simulink model "TB32_A25R_ClampMix"  (R2025a)
settings: Solver=FixedStepDiscrete  StartTime=0  StopTime=TB.t_end  FixedStep=TB.dt  RelTol=1e-3
InitFcn:
  | % 모델과 같은 폴더의 초기화 스크립트를 실행해 P(설계 파라미터)와 TB(시험 조건)를 만든다.
  | run(fullfile(fileparts(get_param(bdroot, 'FileName')), 'TB32_init.m'));
values from neighbouring files (symbols this model uses):
  TB = struct()    [TB32_init.m]    (also in run_TB32.m = evalin('base', 'TB'))
libraries: fl_lib x227, nesl_utility x83
(part 4 of 4)

== system TB32_A25R_ClampMix/StageA_Module3/StageA_Phase6/S2_A_VOUT ==
  note: 스위치 셀: 이상 스위치(R_on, G_off) + 역병렬 바디 다이오드(Vf, R_d) + 출력용량 C_oss
      | 게이트: 전역 태그 "gA_P6_S2" (> 0.5 이면 도통)
  C_oss : fl_lib/Electrical/Electrical Elements/Capacitor  c=Coss F  r=1e-6 Ohm  g=0 1/Ohm  i_specify=off  i_priority=None  i=0 A  i_nominal_specify=off  i_nominal_value=1  i_nominal_unit=A  v_specify=off  v_priority=None  v=0 V  v_nominal_specify=off  v_nominal_value=1  v_nominal_unit=V  vc_specify=off  vc_priority=High  vc=0 V  vc_nominal_specify=off  vc_nominal_value=1  vc_nominal_unit=V
  D_body : fl_lib/Electrical/Electrical Elements/Diode  Vf=Vf V  Ron=Rd Ohm  Goff=Goffd 1/Ohm  i_specify=off  i_priority=None  i=0 A  i_nominal_specify=off  i_nominal_value=1  i_nominal_unit=A  v_specify=off  v_priority=None  v=0 V  v_nominal_specify=off  v_nominal_value=1  v_nominal_unit=V
  Gate_PS : nesl_utility/Simulink-PS Converter  PhysicalDomain=network_engine_domain  SubClassName=ps_input  LeftPortType=input  RightPortType=output  PseudoPeriodic=off  Frequencies=[]  NoiseDistribution=none  NoiseParameters=[]  Unit=1  AffineConversion=off  FilteringAndDerivatives=zero  SimscapeFilterOrder=1  InputFilterTimeConstant=0.001  UdotUserProvided=0
  SW : fl_lib/Electrical/Electrical Elements/Switch  R_closed=Ron Ohm  G_open=Goff 1/Ohm  Threshold=0.5  i_specify=off  i_priority=None  i=0 A  i_nominal_specify=off  i_nominal_value=1  i_nominal_unit=A  v_specify=off  v_priority=None  v=0 V  v_nominal_specify=off  v_nominal_value=1  v_nominal_unit=V
  D : PMIOPort  Side=Left
  S : PMIOPort  Port=2  Side=Right
  wires:
  [gA_P6_S2] -> Gate_PS/1
  connections:
  Gate_PS/RConn1 -- SW/RConn1
  SW/LConn1 -- D/RConn1 -- D_body/RConn1 -- C_oss/LConn1
  SW/RConn2 -- D_body/LConn1 -- S/RConn1 -- C_oss/RConn1

== system TB32_A25R_ClampMix/StageA_Module3/StageA_Phase6/S3_VOUT_B ==
  note: 스위치 셀: 이상 스위치(R_on, G_off) + 역병렬 바디 다이오드(Vf, R_d) + 출력용량 C_oss
      | 게이트: 전역 태그 "gA_P6_S3" (> 0.5 이면 도통)
  C_oss : fl_lib/Electrical/Electrical Elements/Capacitor  c=Coss F  r=1e-6 Ohm  g=0 1/Ohm  i_specify=off  i_priority=None  i=0 A  i_nominal_specify=off  i_nominal_value=1  i_nominal_unit=A  v_specify=off  v_priority=None  v=0 V  v_nominal_specify=off  v_nominal_value=1  v_nominal_unit=V  vc_specify=off  vc_priority=High  vc=0 V  vc_nominal_specify=off  vc_nominal_value=1  vc_nominal_unit=V
  D_body : fl_lib/Electrical/Electrical Elements/Diode  Vf=Vf V  Ron=Rd Ohm  Goff=Goffd 1/Ohm  i_specify=off  i_priority=None  i=0 A  i_nominal_specify=off  i_nominal_value=1  i_nominal_unit=A  v_specify=off  v_priority=None  v=0 V  v_nominal_specify=off  v_nominal_value=1  v_nominal_unit=V
  Gate_PS : nesl_utility/Simulink-PS Converter  PhysicalDomain=network_engine_domain  SubClassName=ps_input  LeftPortType=input  RightPortType=output  PseudoPeriodic=off  Frequencies=[]  NoiseDistribution=none  NoiseParameters=[]  Unit=1  AffineConversion=off  FilteringAndDerivatives=zero  SimscapeFilterOrder=1  InputFilterTimeConstant=0.001  UdotUserProvided=0
  SW : fl_lib/Electrical/Electrical Elements/Switch  R_closed=Ron Ohm  G_open=Goff 1/Ohm  Threshold=0.5  i_specify=off  i_priority=None  i=0 A  i_nominal_specify=off  i_nominal_value=1  i_nominal_unit=A  v_specify=off  v_priority=None  v=0 V  v_nominal_specify=off  v_nominal_value=1  v_nominal_unit=V
  D : PMIOPort  Side=Left
  S : PMIOPort  Port=2  Side=Right
  wires:
  [gA_P6_S3] -> Gate_PS/1
  connections:
  Gate_PS/RConn1 -- SW/RConn1
  SW/LConn1 -- D/RConn1 -- D_body/RConn1 -- C_oss/LConn1
  SW/RConn2 -- D_body/LConn1 -- S/RConn1 -- C_oss/RConn1

== system TB32_A25R_ClampMix/StageA_Module3/StageA_Phase6/S4_B_GND ==
  note: 스위치 셀: 이상 스위치(R_on, G_off) + 역병렬 바디 다이오드(Vf, R_d) + 출력용량 C_oss
      | 게이트: 전역 태그 "gA_P6_S4" (> 0.5 이면 도통)
  C_oss : fl_lib/Electrical/Electrical Elements/Capacitor  c=Coss F  r=1e-6 Ohm  g=0 1/Ohm  i_specify=off  i_priority=None  i=0 A  i_nominal_specify=off  i_nominal_value=1  i_nominal_unit=A  v_specify=off  v_priority=None  v=0 V  v_nominal_specify=off  v_nominal_value=1  v_nominal_unit=V  vc_specify=off  vc_priority=High  vc=0 V  vc_nominal_specify=off  vc_nominal_value=1  vc_nominal_unit=V
  D_body : fl_lib/Electrical/Electrical Elements/Diode  Vf=Vf V  Ron=Rd Ohm  Goff=Goffd 1/Ohm  i_specify=off  i_priority=None  i=0 A  i_nominal_specify=off  i_nominal_value=1  i_nominal_unit=A  v_specify=off  v_priority=None  v=0 V  v_nominal_specify=off  v_nominal_value=1  v_nominal_unit=V
  Gate_PS : nesl_utility/Simulink-PS Converter  PhysicalDomain=network_engine_domain  SubClassName=ps_input  LeftPortType=input  RightPortType=output  PseudoPeriodic=off  Frequencies=[]  NoiseDistribution=none  NoiseParameters=[]  Unit=1  AffineConversion=off  FilteringAndDerivatives=zero  SimscapeFilterOrder=1  InputFilterTimeConstant=0.001  UdotUserProvided=0
  SW : fl_lib/Electrical/Electrical Elements/Switch  R_closed=Ron Ohm  G_open=Goff 1/Ohm  Threshold=0.5  i_specify=off  i_priority=None  i=0 A  i_nominal_specify=off  i_nominal_value=1  i_nominal_unit=A  v_specify=off  v_priority=None  v=0 V  v_nominal_specify=off  v_nominal_value=1  v_nominal_unit=V
  D : PMIOPort  Side=Left
  S : PMIOPort  Port=2  Side=Right
  wires:
  [gA_P6_S4] -> Gate_PS/1
  connections:
  Gate_PS/RConn1 -- SW/RConn1
  SW/LConn1 -- D/RConn1 -- D_body/RConn1 -- C_oss/LConn1
  SW/RConn2 -- D_body/LConn1 -- S/RConn1 -- C_oss/RConn1

== system TB32_A25R_ClampMix/StageA_Module4/StageA_Phase7/S1_VIN_A ==
  note: 스위치 셀: 이상 스위치(R_on, G_off) + 역병렬 바디 다이오드(Vf, R_d) + 출력용량 C_oss
      | 게이트: 전역 태그 "gA_P7_S1" (> 0.5 이면 도통)
  C_oss : fl_lib/Electrical/Electrical Elements/Capacitor  c=Coss F  r=1e-6 Ohm  g=0 1/Ohm  i_specify=off  i_priority=None  i=0 A  i_nominal_specify=off  i_nominal_value=1  i_nominal_unit=A  v_specify=off  v_priority=None  v=0 V  v_nominal_specify=off  v_nominal_value=1  v_nominal_unit=V  vc_specify=off  vc_priority=High  vc=0 V  vc_nominal_specify=off  vc_nominal_value=1  vc_nominal_unit=V
  D_body : fl_lib/Electrical/Electrical Elements/Diode  Vf=Vf V  Ron=Rd Ohm  Goff=Goffd 1/Ohm  i_specify=off  i_priority=None  i=0 A  i_nominal_specify=off  i_nominal_value=1  i_nominal_unit=A  v_specify=off  v_priority=None  v=0 V  v_nominal_specify=off  v_nominal_value=1  v_nominal_unit=V
  Gate_PS : nesl_utility/Simulink-PS Converter  PhysicalDomain=network_engine_domain  SubClassName=ps_input  LeftPortType=input  RightPortType=output  PseudoPeriodic=off  Frequencies=[]  NoiseDistribution=none  NoiseParameters=[]  Unit=1  AffineConversion=off  FilteringAndDerivatives=zero  SimscapeFilterOrder=1  InputFilterTimeConstant=0.001  UdotUserProvided=0
  SW : fl_lib/Electrical/Electrical Elements/Switch  R_closed=Ron Ohm  G_open=Goff 1/Ohm  Threshold=0.5  i_specify=off  i_priority=None  i=0 A  i_nominal_specify=off  i_nominal_value=1  i_nominal_unit=A  v_specify=off  v_priority=None  v=0 V  v_nominal_specify=off  v_nominal_value=1  v_nominal_unit=V
  D : PMIOPort  Side=Left
  S : PMIOPort  Port=2  Side=Right
  wires:
  [gA_P7_S1] -> Gate_PS/1
  connections:
  Gate_PS/RConn1 -- SW/RConn1
  SW/LConn1 -- D/RConn1 -- D_body/RConn1 -- C_oss/LConn1
  SW/RConn2 -- D_body/LConn1 -- S/RConn1 -- C_oss/RConn1

== system TB32_A25R_ClampMix/StageA_Module4/StageA_Phase7/S2_A_VOUT ==
  note: 스위치 셀: 이상 스위치(R_on, G_off) + 역병렬 바디 다이오드(Vf, R_d) + 출력용량 C_oss
      | 게이트: 전역 태그 "gA_P7_S2" (> 0.5 이면 도통)
  C_oss : fl_lib/Electrical/Electrical Elements/Capacitor  c=Coss F  r=1e-6 Ohm  g=0 1/Ohm  i_specify=off  i_priority=None  i=0 A  i_nominal_specify=off  i_nominal_value=1  i_nominal_unit=A  v_specify=off  v_priority=None  v=0 V  v_nominal_specify=off  v_nominal_value=1  v_nominal_unit=V  vc_specify=off  vc_priority=High  vc=0 V  vc_nominal_specify=off  vc_nominal_value=1  vc_nominal_unit=V
  D_body : fl_lib/Electrical/Electrical Elements/Diode  Vf=Vf V  Ron=Rd Ohm  Goff=Goffd 1/Ohm  i_specify=off  i_priority=None  i=0 A  i_nominal_specify=off  i_nominal_value=1  i_nominal_unit=A  v_specify=off  v_priority=None  v=0 V  v_nominal_specify=off  v_nominal_value=1  v_nominal_unit=V
  Gate_PS : nesl_utility/Simulink-PS Converter  PhysicalDomain=network_engine_domain  SubClassName=ps_input  LeftPortType=input  RightPortType=output  PseudoPeriodic=off  Frequencies=[]  NoiseDistribution=none  NoiseParameters=[]  Unit=1  AffineConversion=off  FilteringAndDerivatives=zero  SimscapeFilterOrder=1  InputFilterTimeConstant=0.001  UdotUserProvided=0
  SW : fl_lib/Electrical/Electrical Elements/Switch  R_closed=Ron Ohm  G_open=Goff 1/Ohm  Threshold=0.5  i_specify=off  i_priority=None  i=0 A  i_nominal_specify=off  i_nominal_value=1  i_nominal_unit=A  v_specify=off  v_priority=None  v=0 V  v_nominal_specify=off  v_nominal_value=1  v_nominal_unit=V
  D : PMIOPort  Side=Left
  S : PMIOPort  Port=2  Side=Right
  wires:
  [gA_P7_S2] -> Gate_PS/1
  connections:
  Gate_PS/RConn1 -- SW/RConn1
  SW/LConn1 -- D/RConn1 -- D_body/RConn1 -- C_oss/LConn1
  SW/RConn2 -- D_body/LConn1 -- S/RConn1 -- C_oss/RConn1

== system TB32_A25R_ClampMix/StageA_Module4/StageA_Phase7/S3_VOUT_B ==
  note: 스위치 셀: 이상 스위치(R_on, G_off) + 역병렬 바디 다이오드(Vf, R_d) + 출력용량 C_oss
      | 게이트: 전역 태그 "gA_P7_S3" (> 0.5 이면 도통)
  C_oss : fl_lib/Electrical/Electrical Elements/Capacitor  c=Coss F  r=1e-6 Ohm  g=0 1/Ohm  i_specify=off  i_priority=None  i=0 A  i_nominal_specify=off  i_nominal_value=1  i_nominal_unit=A  v_specify=off  v_priority=None  v=0 V  v_nominal_specify=off  v_nominal_value=1  v_nominal_unit=V  vc_specify=off  vc_priority=High  vc=0 V  vc_nominal_specify=off  vc_nominal_value=1  vc_nominal_unit=V
  D_body : fl_lib/Electrical/Electrical Elements/Diode  Vf=Vf V  Ron=Rd Ohm  Goff=Goffd 1/Ohm  i_specify=off  i_priority=None  i=0 A  i_nominal_specify=off  i_nominal_value=1  i_nominal_unit=A  v_specify=off  v_priority=None  v=0 V  v_nominal_specify=off  v_nominal_value=1  v_nominal_unit=V
  Gate_PS : nesl_utility/Simulink-PS Converter  PhysicalDomain=network_engine_domain  SubClassName=ps_input  LeftPortType=input  RightPortType=output  PseudoPeriodic=off  Frequencies=[]  NoiseDistribution=none  NoiseParameters=[]  Unit=1  AffineConversion=off  FilteringAndDerivatives=zero  SimscapeFilterOrder=1  InputFilterTimeConstant=0.001  UdotUserProvided=0
  SW : fl_lib/Electrical/Electrical Elements/Switch  R_closed=Ron Ohm  G_open=Goff 1/Ohm  Threshold=0.5  i_specify=off  i_priority=None  i=0 A  i_nominal_specify=off  i_nominal_value=1  i_nominal_unit=A  v_specify=off  v_priority=None  v=0 V  v_nominal_specify=off  v_nominal_value=1  v_nominal_unit=V
  D : PMIOPort  Side=Left
  S : PMIOPort  Port=2  Side=Right
  wires:
  [gA_P7_S3] -> Gate_PS/1
  connections:
  Gate_PS/RConn1 -- SW/RConn1
  SW/LConn1 -- D/RConn1 -- D_body/RConn1 -- C_oss/LConn1
  SW/RConn2 -- D_body/LConn1 -- S/RConn1 -- C_oss/RConn1

== system TB32_A25R_ClampMix/StageA_Module4/StageA_Phase7/S4_B_GND ==
  note: 스위치 셀: 이상 스위치(R_on, G_off) + 역병렬 바디 다이오드(Vf, R_d) + 출력용량 C_oss
      | 게이트: 전역 태그 "gA_P7_S4" (> 0.5 이면 도통)
  C_oss : fl_lib/Electrical/Electrical Elements/Capacitor  c=Coss F  r=1e-6 Ohm  g=0 1/Ohm  i_specify=off  i_priority=None  i=0 A  i_nominal_specify=off  i_nominal_value=1  i_nominal_unit=A  v_specify=off  v_priority=None  v=0 V  v_nominal_specify=off  v_nominal_value=1  v_nominal_unit=V  vc_specify=off  vc_priority=High  vc=0 V  vc_nominal_specify=off  vc_nominal_value=1  vc_nominal_unit=V
  D_body : fl_lib/Electrical/Electrical Elements/Diode  Vf=Vf V  Ron=Rd Ohm  Goff=Goffd 1/Ohm  i_specify=off  i_priority=None  i=0 A  i_nominal_specify=off  i_nominal_value=1  i_nominal_unit=A  v_specify=off  v_priority=None  v=0 V  v_nominal_specify=off  v_nominal_value=1  v_nominal_unit=V
  Gate_PS : nesl_utility/Simulink-PS Converter  PhysicalDomain=network_engine_domain  SubClassName=ps_input  LeftPortType=input  RightPortType=output  PseudoPeriodic=off  Frequencies=[]  NoiseDistribution=none  NoiseParameters=[]  Unit=1  AffineConversion=off  FilteringAndDerivatives=zero  SimscapeFilterOrder=1  InputFilterTimeConstant=0.001  UdotUserProvided=0
  SW : fl_lib/Electrical/Electrical Elements/Switch  R_closed=Ron Ohm  G_open=Goff 1/Ohm  Threshold=0.5  i_specify=off  i_priority=None  i=0 A  i_nominal_specify=off  i_nominal_value=1  i_nominal_unit=A  v_specify=off  v_priority=None  v=0 V  v_nominal_specify=off  v_nominal_value=1  v_nominal_unit=V
  D : PMIOPort  Side=Left
  S : PMIOPort  Port=2  Side=Right
  wires:
  [gA_P7_S4] -> Gate_PS/1
  connections:
  Gate_PS/RConn1 -- SW/RConn1
  SW/LConn1 -- D/RConn1 -- D_body/RConn1 -- C_oss/LConn1
  SW/RConn2 -- D_body/LConn1 -- S/RConn1 -- C_oss/RConn1

== system TB32_A25R_ClampMix/StageA_Module4/StageA_Phase8/S1_VIN_A ==
  note: 스위치 셀: 이상 스위치(R_on, G_off) + 역병렬 바디 다이오드(Vf, R_d) + 출력용량 C_oss
      | 게이트: 전역 태그 "gA_P8_S1" (> 0.5 이면 도통)
  C_oss : fl_lib/Electrical/Electrical Elements/Capacitor  c=Coss F  r=1e-6 Ohm  g=0 1/Ohm  i_specify=off  i_priority=None  i=0 A  i_nominal_specify=off  i_nominal_value=1  i_nominal_unit=A  v_specify=off  v_priority=None  v=0 V  v_nominal_specify=off  v_nominal_value=1  v_nominal_unit=V  vc_specify=off  vc_priority=High  vc=0 V  vc_nominal_specify=off  vc_nominal_value=1  vc_nominal_unit=V
  D_body : fl_lib/Electrical/Electrical Elements/Diode  Vf=Vf V  Ron=Rd Ohm  Goff=Goffd 1/Ohm  i_specify=off  i_priority=None  i=0 A  i_nominal_specify=off  i_nominal_value=1  i_nominal_unit=A  v_specify=off  v_priority=None  v=0 V  v_nominal_specify=off  v_nominal_value=1  v_nominal_unit=V
  Gate_PS : nesl_utility/Simulink-PS Converter  PhysicalDomain=network_engine_domain  SubClassName=ps_input  LeftPortType=input  RightPortType=output  PseudoPeriodic=off  Frequencies=[]  NoiseDistribution=none  NoiseParameters=[]  Unit=1  AffineConversion=off  FilteringAndDerivatives=zero  SimscapeFilterOrder=1  InputFilterTimeConstant=0.001  UdotUserProvided=0
  SW : fl_lib/Electrical/Electrical Elements/Switch  R_closed=Ron Ohm  G_open=Goff 1/Ohm  Threshold=0.5  i_specify=off  i_priority=None  i=0 A  i_nominal_specify=off  i_nominal_value=1  i_nominal_unit=A  v_specify=off  v_priority=None  v=0 V  v_nominal_specify=off  v_nominal_value=1  v_nominal_unit=V
  D : PMIOPort  Side=Left
  S : PMIOPort  Port=2  Side=Right
  wires:
  [gA_P8_S1] -> Gate_PS/1
  connections:
  Gate_PS/RConn1 -- SW/RConn1
  SW/LConn1 -- D/RConn1 -- D_body/RConn1 -- C_oss/LConn1
  SW/RConn2 -- D_body/LConn1 -- S/RConn1 -- C_oss/RConn1

== system TB32_A25R_ClampMix/StageA_Module4/StageA_Phase8/S2_A_VOUT ==
  note: 스위치 셀: 이상 스위치(R_on, G_off) + 역병렬 바디 다이오드(Vf, R_d) + 출력용량 C_oss
      | 게이트: 전역 태그 "gA_P8_S2" (> 0.5 이면 도통)
  C_oss : fl_lib/Electrical/Electrical Elements/Capacitor  c=Coss F  r=1e-6 Ohm  g=0 1/Ohm  i_specify=off  i_priority=None  i=0 A  i_nominal_specify=off  i_nominal_value=1  i_nominal_unit=A  v_specify=off  v_priority=None  v=0 V  v_nominal_specify=off  v_nominal_value=1  v_nominal_unit=V  vc_specify=off  vc_priority=High  vc=0 V  vc_nominal_specify=off  vc_nominal_value=1  vc_nominal_unit=V
  D_body : fl_lib/Electrical/Electrical Elements/Diode  Vf=Vf V  Ron=Rd Ohm  Goff=Goffd 1/Ohm  i_specify=off  i_priority=None  i=0 A  i_nominal_specify=off  i_nominal_value=1  i_nominal_unit=A  v_specify=off  v_priority=None  v=0 V  v_nominal_specify=off  v_nominal_value=1  v_nominal_unit=V
  Gate_PS : nesl_utility/Simulink-PS Converter  PhysicalDomain=network_engine_domain  SubClassName=ps_input  LeftPortType=input  RightPortType=output  PseudoPeriodic=off  Frequencies=[]  NoiseDistribution=none  NoiseParameters=[]  Unit=1  AffineConversion=off  FilteringAndDerivatives=zero  SimscapeFilterOrder=1  InputFilterTimeConstant=0.001  UdotUserProvided=0
  SW : fl_lib/Electrical/Electrical Elements/Switch  R_closed=Ron Ohm  G_open=Goff 1/Ohm  Threshold=0.5  i_specify=off  i_priority=None  i=0 A  i_nominal_specify=off  i_nominal_value=1  i_nominal_unit=A  v_specify=off  v_priority=None  v=0 V  v_nominal_specify=off  v_nominal_value=1  v_nominal_unit=V
  D : PMIOPort  Side=Left
  S : PMIOPort  Port=2  Side=Right
  wires:
  [gA_P8_S2] -> Gate_PS/1
  connections:
  Gate_PS/RConn1 -- SW/RConn1
  SW/LConn1 -- D/RConn1 -- D_body/RConn1 -- C_oss/LConn1
  SW/RConn2 -- D_body/LConn1 -- S/RConn1 -- C_oss/RConn1

== system TB32_A25R_ClampMix/StageA_Module4/StageA_Phase8/S3_VOUT_B ==
  note: 스위치 셀: 이상 스위치(R_on, G_off) + 역병렬 바디 다이오드(Vf, R_d) + 출력용량 C_oss
      | 게이트: 전역 태그 "gA_P8_S3" (> 0.5 이면 도통)
  C_oss : fl_lib/Electrical/Electrical Elements/Capacitor  c=Coss F  r=1e-6 Ohm  g=0 1/Ohm  i_specify=off  i_priority=None  i=0 A  i_nominal_specify=off  i_nominal_value=1  i_nominal_unit=A  v_specify=off  v_priority=None  v=0 V  v_nominal_specify=off  v_nominal_value=1  v_nominal_unit=V  vc_specify=off  vc_priority=High  vc=0 V  vc_nominal_specify=off  vc_nominal_value=1  vc_nominal_unit=V
  D_body : fl_lib/Electrical/Electrical Elements/Diode  Vf=Vf V  Ron=Rd Ohm  Goff=Goffd 1/Ohm  i_specify=off  i_priority=None  i=0 A  i_nominal_specify=off  i_nominal_value=1  i_nominal_unit=A  v_specify=off  v_priority=None  v=0 V  v_nominal_specify=off  v_nominal_value=1  v_nominal_unit=V
  Gate_PS : nesl_utility/Simulink-PS Converter  PhysicalDomain=network_engine_domain  SubClassName=ps_input  LeftPortType=input  RightPortType=output  PseudoPeriodic=off  Frequencies=[]  NoiseDistribution=none  NoiseParameters=[]  Unit=1  AffineConversion=off  FilteringAndDerivatives=zero  SimscapeFilterOrder=1  InputFilterTimeConstant=0.001  UdotUserProvided=0
  SW : fl_lib/Electrical/Electrical Elements/Switch  R_closed=Ron Ohm  G_open=Goff 1/Ohm  Threshold=0.5  i_specify=off  i_priority=None  i=0 A  i_nominal_specify=off  i_nominal_value=1  i_nominal_unit=A  v_specify=off  v_priority=None  v=0 V  v_nominal_specify=off  v_nominal_value=1  v_nominal_unit=V
  D : PMIOPort  Side=Left
  S : PMIOPort  Port=2  Side=Right
  wires:
  [gA_P8_S3] -> Gate_PS/1
  connections:
  Gate_PS/RConn1 -- SW/RConn1
  SW/LConn1 -- D/RConn1 -- D_body/RConn1 -- C_oss/LConn1
  SW/RConn2 -- D_body/LConn1 -- S/RConn1 -- C_oss/RConn1

== system TB32_A25R_ClampMix/StageA_Module4/StageA_Phase8/S4_B_GND ==
  note: 스위치 셀: 이상 스위치(R_on, G_off) + 역병렬 바디 다이오드(Vf, R_d) + 출력용량 C_oss
      | 게이트: 전역 태그 "gA_P8_S4" (> 0.5 이면 도통)
  C_oss : fl_lib/Electrical/Electrical Elements/Capacitor  c=Coss F  r=1e-6 Ohm  g=0 1/Ohm  i_specify=off  i_priority=None  i=0 A  i_nominal_specify=off  i_nominal_value=1  i_nominal_unit=A  v_specify=off  v_priority=None  v=0 V  v_nominal_specify=off  v_nominal_value=1  v_nominal_unit=V  vc_specify=off  vc_priority=High  vc=0 V  vc_nominal_specify=off  vc_nominal_value=1  vc_nominal_unit=V
  D_body : fl_lib/Electrical/Electrical Elements/Diode  Vf=Vf V  Ron=Rd Ohm  Goff=Goffd 1/Ohm  i_specify=off  i_priority=None  i=0 A  i_nominal_specify=off  i_nominal_value=1  i_nominal_unit=A  v_specify=off  v_priority=None  v=0 V  v_nominal_specify=off  v_nominal_value=1  v_nominal_unit=V
  Gate_PS : nesl_utility/Simulink-PS Converter  PhysicalDomain=network_engine_domain  SubClassName=ps_input  LeftPortType=input  RightPortType=output  PseudoPeriodic=off  Frequencies=[]  NoiseDistribution=none  NoiseParameters=[]  Unit=1  AffineConversion=off  FilteringAndDerivatives=zero  SimscapeFilterOrder=1  InputFilterTimeConstant=0.001  UdotUserProvided=0
  SW : fl_lib/Electrical/Electrical Elements/Switch  R_closed=Ron Ohm  G_open=Goff 1/Ohm  Threshold=0.5  i_specify=off  i_priority=None  i=0 A  i_nominal_specify=off  i_nominal_value=1  i_nominal_unit=A  v_specify=off  v_priority=None  v=0 V  v_nominal_specify=off  v_nominal_value=1  v_nominal_unit=V
  D : PMIOPort  Side=Left
  S : PMIOPort  Port=2  Side=Right
  wires:
  [gA_P8_S4] -> Gate_PS/1
  connections:
  Gate_PS/RConn1 -- SW/RConn1
  SW/LConn1 -- D/RConn1 -- D_body/RConn1 -- C_oss/LConn1
  SW/RConn2 -- D_body/LConn1 -- S/RConn1 -- C_oss/RConn1

== system TB32_A25R_ClampMix/StageC_Regulated/Primary_Bridge/Q1_leg1_high ==
  note: 스위치 셀: 이상 스위치(R_on, G_off) + 역병렬 바디 다이오드(Vf, R_d) + 출력용량 C_oss
      | 게이트: 전역 태그 "gC_Q1" (> 0.5 이면 도통)
  C_oss : fl_lib/Electrical/Electrical Elements/Capacitor  c=Coss F  r=1e-6 Ohm  g=0 1/Ohm  i_specify=off  i_priority=None  i=0 A  i_nominal_specify=off  i_nominal_value=1  i_nominal_unit=A  v_specify=off  v_priority=None  v=0 V  v_nominal_specify=off  v_nominal_value=1  v_nominal_unit=V  vc_specify=off  vc_priority=High  vc=0 V  vc_nominal_specify=off  vc_nominal_value=1  vc_nominal_unit=V
  D_body : fl_lib/Electrical/Electrical Elements/Diode  Vf=Vf V  Ron=Rd Ohm  Goff=Goffd 1/Ohm  i_specify=off  i_priority=None  i=0 A  i_nominal_specify=off  i_nominal_value=1  i_nominal_unit=A  v_specify=off  v_priority=None  v=0 V  v_nominal_specify=off  v_nominal_value=1  v_nominal_unit=V
  Gate_PS : nesl_utility/Simulink-PS Converter  PhysicalDomain=network_engine_domain  SubClassName=ps_input  LeftPortType=input  RightPortType=output  PseudoPeriodic=off  Frequencies=[]  NoiseDistribution=none  NoiseParameters=[]  Unit=1  AffineConversion=off  FilteringAndDerivatives=zero  SimscapeFilterOrder=1  InputFilterTimeConstant=0.001  UdotUserProvided=0
  SW : fl_lib/Electrical/Electrical Elements/Switch  R_closed=Ron Ohm  G_open=Goff 1/Ohm  Threshold=0.5  i_specify=off  i_priority=None  i=0 A  i_nominal_specify=off  i_nominal_value=1  i_nominal_unit=A  v_specify=off  v_priority=None  v=0 V  v_nominal_specify=off  v_nominal_value=1  v_nominal_unit=V
  D : PMIOPort  Side=Left
  S : PMIOPort  Port=2  Side=Right
  wires:
  [gC_Q1] -> Gate_PS/1
  connections:
  Gate_PS/RConn1 -- SW/RConn1
  SW/LConn1 -- D/RConn1 -- D_body/RConn1 -- C_oss/LConn1
  SW/RConn2 -- D_body/LConn1 -- S/RConn1 -- C_oss/RConn1

== system TB32_A25R_ClampMix/StageC_Regulated/Primary_Bridge/Q2_leg1_low ==
  note: 스위치 셀: 이상 스위치(R_on, G_off) + 역병렬 바디 다이오드(Vf, R_d) + 출력용량 C_oss
      | 게이트: 전역 태그 "gC_Q2" (> 0.5 이면 도통)
  C_oss : fl_lib/Electrical/Electrical Elements/Capacitor  c=Coss F  r=1e-6 Ohm  g=0 1/Ohm  i_specify=off  i_priority=None  i=0 A  i_nominal_specify=off  i_nominal_value=1  i_nominal_unit=A  v_specify=off  v_priority=None  v=0 V  v_nominal_specify=off  v_nominal_value=1  v_nominal_unit=V  vc_specify=off  vc_priority=High  vc=0 V  vc_nominal_specify=off  vc_nominal_value=1  vc_nominal_unit=V
  D_body : fl_lib/Electrical/Electrical Elements/Diode  Vf=Vf V  Ron=Rd Ohm  Goff=Goffd 1/Ohm  i_specify=off  i_priority=None  i=0 A  i_nominal_specify=off  i_nominal_value=1  i_nominal_unit=A  v_specify=off  v_priority=None  v=0 V  v_nominal_specify=off  v_nominal_value=1  v_nominal_unit=V
  Gate_PS : nesl_utility/Simulink-PS Converter  PhysicalDomain=network_engine_domain  SubClassName=ps_input  LeftPortType=input  RightPortType=output  PseudoPeriodic=off  Frequencies=[]  NoiseDistribution=none  NoiseParameters=[]  Unit=1  AffineConversion=off  FilteringAndDerivatives=zero  SimscapeFilterOrder=1  InputFilterTimeConstant=0.001  UdotUserProvided=0
  SW : fl_lib/Electrical/Electrical Elements/Switch  R_closed=Ron Ohm  G_open=Goff 1/Ohm  Threshold=0.5  i_specify=off  i_priority=None  i=0 A  i_nominal_specify=off  i_nominal_value=1  i_nominal_unit=A  v_specify=off  v_priority=None  v=0 V  v_nominal_specify=off  v_nominal_value=1  v_nominal_unit=V
  D : PMIOPort  Side=Left
  S : PMIOPort  Port=2  Side=Right
  wires:
  [gC_Q2] -> Gate_PS/1
  connections:
  Gate_PS/RConn1 -- SW/RConn1
  SW/LConn1 -- D/RConn1 -- D_body/RConn1 -- C_oss/LConn1
  SW/RConn2 -- D_body/LConn1 -- S/RConn1 -- C_oss/RConn1

== system TB32_A25R_ClampMix/StageC_Regulated/Primary_Bridge/Q3_leg2_high ==
  note: 스위치 셀: 이상 스위치(R_on, G_off) + 역병렬 바디 다이오드(Vf, R_d) + 출력용량 C_oss
      | 게이트: 전역 태그 "gC_Q3" (> 0.5 이면 도통)
  C_oss : fl_lib/Electrical/Electrical Elements/Capacitor  c=Coss F  r=1e-6 Ohm  g=0 1/Ohm  i_specify=off  i_priority=None  i=0 A  i_nominal_specify=off  i_nominal_value=1  i_nominal_unit=A  v_specify=off  v_priority=None  v=0 V  v_nominal_specify=off  v_nominal_value=1  v_nominal_unit=V  vc_specify=off  vc_priority=High  vc=0 V  vc_nominal_specify=off  vc_nominal_value=1  vc_nominal_unit=V
  D_body : fl_lib/Electrical/Electrical Elements/Diode  Vf=Vf V  Ron=Rd Ohm  Goff=Goffd 1/Ohm  i_specify=off  i_priority=None  i=0 A  i_nominal_specify=off  i_nominal_value=1  i_nominal_unit=A  v_specify=off  v_priority=None  v=0 V  v_nominal_specify=off  v_nominal_value=1  v_nominal_unit=V
  Gate_PS : nesl_utility/Simulink-PS Converter  PhysicalDomain=network_engine_domain  SubClassName=ps_input  LeftPortType=input  RightPortType=output  PseudoPeriodic=off  Frequencies=[]  NoiseDistribution=none  NoiseParameters=[]  Unit=1  AffineConversion=off  FilteringAndDerivatives=zero  SimscapeFilterOrder=1  InputFilterTimeConstant=0.001  UdotUserProvided=0
  SW : fl_lib/Electrical/Electrical Elements/Switch  R_closed=Ron Ohm  G_open=Goff 1/Ohm  Threshold=0.5  i_specify=off  i_priority=None  i=0 A  i_nominal_specify=off  i_nominal_value=1  i_nominal_unit=A  v_specify=off  v_priority=None  v=0 V  v_nominal_specify=off  v_nominal_value=1  v_nominal_unit=V
  D : PMIOPort  Side=Left
  S : PMIOPort  Port=2  Side=Right
  wires:
  [gC_Q3] -> Gate_PS/1
  connections:
  Gate_PS/RConn1 -- SW/RConn1
  SW/LConn1 -- D/RConn1 -- D_body/RConn1 -- C_oss/LConn1
  SW/RConn2 -- D_body/LConn1 -- S/RConn1 -- C_oss/RConn1

== system TB32_A25R_ClampMix/StageC_Regulated/Primary_Bridge/Q4_leg2_low ==
  note: 스위치 셀: 이상 스위치(R_on, G_off) + 역병렬 바디 다이오드(Vf, R_d) + 출력용량 C_oss
      | 게이트: 전역 태그 "gC_Q4" (> 0.5 이면 도통)
  C_oss : fl_lib/Electrical/Electrical Elements/Capacitor  c=Coss F  r=1e-6 Ohm  g=0 1/Ohm  i_specify=off  i_priority=None  i=0 A  i_nominal_specify=off  i_nominal_value=1  i_nominal_unit=A  v_specify=off  v_priority=None  v=0 V  v_nominal_specify=off  v_nominal_value=1  v_nominal_unit=V  vc_specify=off  vc_priority=High  vc=0 V  vc_nominal_specify=off  vc_nominal_value=1  vc_nominal_unit=V
  D_body : fl_lib/Electrical/Electrical Elements/Diode  Vf=Vf V  Ron=Rd Ohm  Goff=Goffd 1/Ohm  i_specify=off  i_priority=None  i=0 A  i_nominal_specify=off  i_nominal_value=1  i_nominal_unit=A  v_specify=off  v_priority=None  v=0 V  v_nominal_specify=off  v_nominal_value=1  v_nominal_unit=V
  Gate_PS : nesl_utility/Simulink-PS Converter  PhysicalDomain=network_engine_domain  SubClassName=ps_input  LeftPortType=input  RightPortType=output  PseudoPeriodic=off  Frequencies=[]  NoiseDistribution=none  NoiseParameters=[]  Unit=1  AffineConversion=off  FilteringAndDerivatives=zero  SimscapeFilterOrder=1  InputFilterTimeConstant=0.001  UdotUserProvided=0
  SW : fl_lib/Electrical/Electrical Elements/Switch  R_closed=Ron Ohm  G_open=Goff 1/Ohm  Threshold=0.5  i_specify=off  i_priority=None  i=0 A  i_nominal_specify=off  i_nominal_value=1  i_nominal_unit=A  v_specify=off  v_priority=None  v=0 V  v_nominal_specify=off  v_nominal_value=1  v_nominal_unit=V
  D : PMIOPort  Side=Left
  S : PMIOPort  Port=2  Side=Right
  wires:
  [gC_Q4] -> Gate_PS/1
  connections:
  Gate_PS/RConn1 -- SW/RConn1
  SW/LConn1 -- D/RConn1 -- D_body/RConn1 -- C_oss/LConn1
  SW/RConn2 -- D_body/LConn1 -- S/RConn1 -- C_oss/RConn1

== system TB32_A25R_ClampMix/StageC_Regulated/Secondary_Bridge/S1_leg1_high ==
  note: 스위치 셀: 이상 스위치(R_on, G_off) + 역병렬 바디 다이오드(Vf, R_d) + 출력용량 C_oss
      | 게이트: 전역 태그 "gC_S1" (> 0.5 이면 도통)
  C_oss : fl_lib/Electrical/Electrical Elements/Capacitor  c=Coss F  r=1e-6 Ohm  g=0 1/Ohm  i_specify=off  i_priority=None  i=0 A  i_nominal_specify=off  i_nominal_value=1  i_nominal_unit=A  v_specify=off  v_priority=None  v=0 V  v_nominal_specify=off  v_nominal_value=1  v_nominal_unit=V  vc_specify=off  vc_priority=High  vc=0 V  vc_nominal_specify=off  vc_nominal_value=1  vc_nominal_unit=V
  D_body : fl_lib/Electrical/Electrical Elements/Diode  Vf=Vf V  Ron=Rd Ohm  Goff=Goffd 1/Ohm  i_specify=off  i_priority=None  i=0 A  i_nominal_specify=off  i_nominal_value=1  i_nominal_unit=A  v_specify=off  v_priority=None  v=0 V  v_nominal_specify=off  v_nominal_value=1  v_nominal_unit=V
  Gate_PS : nesl_utility/Simulink-PS Converter  PhysicalDomain=network_engine_domain  SubClassName=ps_input  LeftPortType=input  RightPortType=output  PseudoPeriodic=off  Frequencies=[]  NoiseDistribution=none  NoiseParameters=[]  Unit=1  AffineConversion=off  FilteringAndDerivatives=zero  SimscapeFilterOrder=1  InputFilterTimeConstant=0.001  UdotUserProvided=0
  SW : fl_lib/Electrical/Electrical Elements/Switch  R_closed=Ron Ohm  G_open=Goff 1/Ohm  Threshold=0.5  i_specify=off  i_priority=None  i=0 A  i_nominal_specify=off  i_nominal_value=1  i_nominal_unit=A  v_specify=off  v_priority=None  v=0 V  v_nominal_specify=off  v_nominal_value=1  v_nominal_unit=V
  D : PMIOPort  Side=Left
  S : PMIOPort  Port=2  Side=Right
  wires:
  [gC_S1] -> Gate_PS/1
  connections:
  Gate_PS/RConn1 -- SW/RConn1
  SW/LConn1 -- D/RConn1 -- D_body/RConn1 -- C_oss/LConn1
  SW/RConn2 -- D_body/LConn1 -- S/RConn1 -- C_oss/RConn1

== system TB32_A25R_ClampMix/StageC_Regulated/Secondary_Bridge/S2_leg1_low ==
  note: 스위치 셀: 이상 스위치(R_on, G_off) + 역병렬 바디 다이오드(Vf, R_d) + 출력용량 C_oss
      | 게이트: 전역 태그 "gC_S2" (> 0.5 이면 도통)
  C_oss : fl_lib/Electrical/Electrical Elements/Capacitor  c=Coss F  r=1e-6 Ohm  g=0 1/Ohm  i_specify=off  i_priority=None  i=0 A  i_nominal_specify=off  i_nominal_value=1  i_nominal_unit=A  v_specify=off  v_priority=None  v=0 V  v_nominal_specify=off  v_nominal_value=1  v_nominal_unit=V  vc_specify=off  vc_priority=High  vc=0 V  vc_nominal_specify=off  vc_nominal_value=1  vc_nominal_unit=V
  D_body : fl_lib/Electrical/Electrical Elements/Diode  Vf=Vf V  Ron=Rd Ohm  Goff=Goffd 1/Ohm  i_specify=off  i_priority=None  i=0 A  i_nominal_specify=off  i_nominal_value=1  i_nominal_unit=A  v_specify=off  v_priority=None  v=0 V  v_nominal_specify=off  v_nominal_value=1  v_nominal_unit=V
  Gate_PS : nesl_utility/Simulink-PS Converter  PhysicalDomain=network_engine_domain  SubClassName=ps_input  LeftPortType=input  RightPortType=output  PseudoPeriodic=off  Frequencies=[]  NoiseDistribution=none  NoiseParameters=[]  Unit=1  AffineConversion=off  FilteringAndDerivatives=zero  SimscapeFilterOrder=1  InputFilterTimeConstant=0.001  UdotUserProvided=0
  SW : fl_lib/Electrical/Electrical Elements/Switch  R_closed=Ron Ohm  G_open=Goff 1/Ohm  Threshold=0.5  i_specify=off  i_priority=None  i=0 A  i_nominal_specify=off  i_nominal_value=1  i_nominal_unit=A  v_specify=off  v_priority=None  v=0 V  v_nominal_specify=off  v_nominal_value=1  v_nominal_unit=V
  D : PMIOPort  Side=Left
  S : PMIOPort  Port=2  Side=Right
  wires:
  [gC_S2] -> Gate_PS/1
  connections:
  Gate_PS/RConn1 -- SW/RConn1
  SW/LConn1 -- D/RConn1 -- D_body/RConn1 -- C_oss/LConn1
  SW/RConn2 -- D_body/LConn1 -- S/RConn1 -- C_oss/RConn1

== system TB32_A25R_ClampMix/StageC_Regulated/Secondary_Bridge/S3_leg2_high ==
  note: 스위치 셀: 이상 스위치(R_on, G_off) + 역병렬 바디 다이오드(Vf, R_d) + 출력용량 C_oss
      | 게이트: 전역 태그 "gC_S3" (> 0.5 이면 도통)
  C_oss : fl_lib/Electrical/Electrical Elements/Capacitor  c=Coss F  r=1e-6 Ohm  g=0 1/Ohm  i_specify=off  i_priority=None  i=0 A  i_nominal_specify=off  i_nominal_value=1  i_nominal_unit=A  v_specify=off  v_priority=None  v=0 V  v_nominal_specify=off  v_nominal_value=1  v_nominal_unit=V  vc_specify=off  vc_priority=High  vc=0 V  vc_nominal_specify=off  vc_nominal_value=1  vc_nominal_unit=V
  D_body : fl_lib/Electrical/Electrical Elements/Diode  Vf=Vf V  Ron=Rd Ohm  Goff=Goffd 1/Ohm  i_specify=off  i_priority=None  i=0 A  i_nominal_specify=off  i_nominal_value=1  i_nominal_unit=A  v_specify=off  v_priority=None  v=0 V  v_nominal_specify=off  v_nominal_value=1  v_nominal_unit=V
  Gate_PS : nesl_utility/Simulink-PS Converter  PhysicalDomain=network_engine_domain  SubClassName=ps_input  LeftPortType=input  RightPortType=output  PseudoPeriodic=off  Frequencies=[]  NoiseDistribution=none  NoiseParameters=[]  Unit=1  AffineConversion=off  FilteringAndDerivatives=zero  SimscapeFilterOrder=1  InputFilterTimeConstant=0.001  UdotUserProvided=0
  SW : fl_lib/Electrical/Electrical Elements/Switch  R_closed=Ron Ohm  G_open=Goff 1/Ohm  Threshold=0.5  i_specify=off  i_priority=None  i=0 A  i_nominal_specify=off  i_nominal_value=1  i_nominal_unit=A  v_specify=off  v_priority=None  v=0 V  v_nominal_specify=off  v_nominal_value=1  v_nominal_unit=V
  D : PMIOPort  Side=Left
  S : PMIOPort  Port=2  Side=Right
  wires:
  [gC_S3] -> Gate_PS/1
  connections:
  Gate_PS/RConn1 -- SW/RConn1
  SW/LConn1 -- D/RConn1 -- D_body/RConn1 -- C_oss/LConn1
  SW/RConn2 -- D_body/LConn1 -- S/RConn1 -- C_oss/RConn1

== system TB32_A25R_ClampMix/StageC_Regulated/Secondary_Bridge/S4_leg2_low ==
  note: 스위치 셀: 이상 스위치(R_on, G_off) + 역병렬 바디 다이오드(Vf, R_d) + 출력용량 C_oss
      | 게이트: 전역 태그 "gC_S4" (> 0.5 이면 도통)
  C_oss : fl_lib/Electrical/Electrical Elements/Capacitor  c=Coss F  r=1e-6 Ohm  g=0 1/Ohm  i_specify=off  i_priority=None  i=0 A  i_nominal_specify=off  i_nominal_value=1  i_nominal_unit=A  v_specify=off  v_priority=None  v=0 V  v_nominal_specify=off  v_nominal_value=1  v_nominal_unit=V  vc_specify=off  vc_priority=High  vc=0 V  vc_nominal_specify=off  vc_nominal_value=1  vc_nominal_unit=V
  D_body : fl_lib/Electrical/Electrical Elements/Diode  Vf=Vf V  Ron=Rd Ohm  Goff=Goffd 1/Ohm  i_specify=off  i_priority=None  i=0 A  i_nominal_specify=off  i_nominal_value=1  i_nominal_unit=A  v_specify=off  v_priority=None  v=0 V  v_nominal_specify=off  v_nominal_value=1  v_nominal_unit=V
  Gate_PS : nesl_utility/Simulink-PS Converter  PhysicalDomain=network_engine_domain  SubClassName=ps_input  LeftPortType=input  RightPortType=output  PseudoPeriodic=off  Frequencies=[]  NoiseDistribution=none  NoiseParameters=[]  Unit=1  AffineConversion=off  FilteringAndDerivatives=zero  SimscapeFilterOrder=1  InputFilterTimeConstant=0.001  UdotUserProvided=0
  SW : fl_lib/Electrical/Electrical Elements/Switch  R_closed=Ron Ohm  G_open=Goff 1/Ohm  Threshold=0.5  i_specify=off  i_priority=None  i=0 A  i_nominal_specify=off  i_nominal_value=1  i_nominal_unit=A  v_specify=off  v_priority=None  v=0 V  v_nominal_specify=off  v_nominal_value=1  v_nominal_unit=V
  D : PMIOPort  Side=Left
  S : PMIOPort  Port=2  Side=Right
  wires:
  [gC_S4] -> Gate_PS/1
  connections:
  Gate_PS/RConn1 -- SW/RConn1
  SW/LConn1 -- D/RConn1 -- D_body/RConn1 -- C_oss/LConn1
  SW/RConn2 -- D_body/LConn1 -- S/RConn1 -- C_oss/RConn1

== matlab function TB32_A25R_ClampMix/Gate_StageA/StageA_ZCP_Gate ==
  data: t input; g output; iC input; prm input; chg input; en input; off input; st_out output; mg_out output
function [g, st_out, mg_out] = prism_gate_stageA_zcpf(t, iC, prm, chg, en, off)
%#codegen
%PRISM_GATE_STAGEA_ZCPF  Stage A 4모듈 게이트(TB22의 zcpm) + 모듈 고장 처리(고장 모듈을 관리기 후보에서 뺌). TB24부터.
%
%   prism_gate_stageA_zcpm.m(E28)과 같은 순서·조건에 다음을 더했다(검증 코드 E30 model_stage_a.mgr_fault·일반화한 mgr_step과 같음).
%     0) 모듈 고장: 간격 번호 kk = n_f(prm(23))에서 모듈 fm(prm(22), 1–4, 0이면 없음)의 고장을 처리한다.
%        그 모듈 위상의 구간을 바로 0(네 스위치 끔)으로 하고 영구히 막는다. 건전 모듈 목록에서 빼고, 동작 중이었으면
%        동작 수를 1 줄인다. 동작 모듈이 0이 되면 다음 건전 모듈을 바로 두 위상으로 시작하고 추가 막는 시간 n_lock을 건다.
%     관리기는 건전 모듈 가운데 번호가 작은 것부터 동작시킨다(모듈 m의 순위 rk(m) ≤ 동작 수면 동작). 고장이 없으면
%     건전 모듈 = 1–4, 순위 = 번호라 zcpm과 같다.
%   그 밖의 설명은 prism_gate_stageA_zcpm.m을 본다.
%
%   입력  t, iC, chg, en, off: zcpm과 같다.
%         prm  zcpm의 21개 + [fm n_f] = 23개(fm: 고장 모듈 1–4, 0이면 고장 없음, n_f: 고장 간격 번호, 첫 호출 = 0)
%   출력  g 32×1, st_out 8×1, mg_out 8×1 [동작 수; 모듈 1–4 모드(고장 모듈은 0); If; 취소 수]

N = 8; NM = 4;
persistent st nxt tmr oncnt armed det psign mmode tlow blk If Ifm nact tdn tlock mcancel kstep kk fl
ndead = prm(2); nmin = prm(3); nmax = prm(4); ndet = prm(5); ithr = prm(6); nnom = prm(7);
Ioff = prm(8); Ion = prm(9); Ipkon = prm(10); a = prm(11); ndwell = prm(12);
Imup = prm(13); Imdn = prm(14); Ipkm = prm(15); ndwm = prm(16); nlock = prm(17); n0 = prm(18); If0 = prm(19); nhold = prm(20); am = prm(21);
fm = prm(22); nf = prm(23);
if isempty(st)
    st = zeros(N, 1); nxt = ones(N, 1); tmr = -off(:); oncnt = zeros(N, 1);
    armed = zeros(N, 1); det = zeros(N, 1); psign = zeros(N, 1);
    nact = n0; If = If0; Ifm = zeros(NM, 1); mmode = zeros(NM, 1); tlow = zeros(NM, 1); blk = zeros(N, 1);
    tdn = 0; tlock = 0; mcancel = 0; kstep = 0; kk = 0; fl = zeros(NM, 1);
    for m = 1:NM
        if m <= n0
            mmode(m) = 2; Ifm(m) = If0/n0;
        else
            blk(2*m - 1) = 1; blk(2*m) = 1;
        end
    end
end

% ---- 0) 모듈 고장(E30 mgr_fault) ---------------------------------------------------------------------------
if fm > 0 && kk == nf && fl(fm) < 0.5
    [hl, nh, rk] = healthy(fl, NM);
    was = rk(fm) <= nact;
    fl(fm) = 1;
    if was
        nact = nact - 1;
    end
    mmode(fm) = 0; tlow(fm) = 0; blk(2*fm - 1) = 1; blk(2*fm) = 1;
    for k = 2*fm - 1:2*fm
        st(k) = 0; tmr(k) = 0; armed(k) = 0; det(k) = 0; oncnt(k) = 0;
    end
    [hl, nh, rk] = healthy(fl, NM);
    if nact == 0 && nh > 0
        x = hl(1);
        mmode(x) = 2; tlow(x) = 0; blk(2*x - 1) = 0; blk(2*x) = 0;
        nact = 1; tdn = 0; tlock = nlock;
    end
end
[hl, nh, rk] = healthy(fl, NM);

% ---- 1) 출력전류와 필터 ---------------------------------------------------------------------------------
io = 0; iom = zeros(NM, 1);
for k = 1:N
    x = 0;
    if st(k) == 1
        x = iC(k);
    elseif st(k) == 2
        x = -iC(k);
    end
    io = io + x;
    m = ceil(k/2); iom(m) = iom(m) + x;
end
If = If + (io - If)*am;                           % 모듈 수 판단용(느린 필터)
Ifm = Ifm + (iom - Ifm)*a;

% ---- 2)·3) 모듈 관리 --------------------------------------------------------------------------------------
pk = 0;
for k = 1:N
    if mmode(ceil(k/2)) ~= 0 && abs(iC(k)) > pk
        pk = abs(iC(k));
    end
end
Ia = abs(If);
inhold = kstep < nhold;                              % 시작 유지 구간: 모듈 수를 바꾸지 않는다
if inhold
    kstep = kstep + 1;
end
if tlock > 0
    tlock = tlock - 1;
end
up = chg > 0.5 || (tlock == 0 && (Ia > nact*Imup || pk > Ipkm));
if inhold
    tdn = 0;
elseif nact < nh && up
    if chg > 0.5
        nnew = nh;
    else
        nnew = min(nh, max(nact + 1, ceil(Ia/Imup)));
    end
    for j = nact + 1:nnew
        m = hl(j);
        if mmode(m) == 5
            mcancel = mcancel + 1;
        end
        mmode(m) = 2; tlow(m) = 0; blk(2*m - 1) = 0; blk(2*m) = 0;
    end
    nact = nnew; tdn = 0; tlock = nlock;
elseif chg < 0.5 && nact > 1
    ndn = max(1, ceil(Ia/Imdn));
    if ndn < nact, tdn = tdn + 1; else, tdn = 0; end
    if tdn >= ndwm
        for j = ndn + 1:nact
            mmode(hl(j)) = 5;
        end
        for j = 1:ndn                                % 남는 모듈은 두 위상으로
            m = hl(j);
            if mmode(m) == 1 || mmode(m) == 3
                mmode(m) = 2; blk(2*m) = 0;
            end
            tlow(m) = 0;
        end
        nact = ndn; tdn = 0;
    end
else
    tdn = 0;
end

% ---- 4) 모듈별 위상 셰딩, 멈추는 모듈 ----------------------------------------------------------------------
for m = 1:NM
    kp = 2*m - 1; ks = 2*m;
    if rk(m) <= nact
        ret = abs(Ifm(m)) > Ion || abs(iC(kp)) > Ipkon;
        if mmode(m) == 2
            if abs(Ifm(m)) < Ioff, tlow(m) = tlow(m) + 1; else, tlow(m) = 0; end
            if tlow(m) >= ndwell, mmode(m) = 3; end
        elseif mmode(m) == 3
            if ret
                mmode(m) = 2; tlow(m) = 0;
            elseif st(ks) == 0
                blk(ks) = 1; mmode(m) = 1;
            end
        elseif mmode(m) == 1
            if ret
                blk(ks) = 0; mmode(m) = 2; tlow(m) = 0;
            end
        end
    elseif mmode(m) == 5
        if st(kp) == 0, blk(kp) = 1; end
        if st(ks) == 0, blk(ks) = 1; end
        if blk(kp) > 0.5 && blk(ks) > 0.5, mmode(m) = 0; end
    end
end

% ---- 5) 영교차 추종(방향 반전 처리, 막힌 위상은 시작하지 않음) ----------------------------------------------
for k = 1:N
    if en(k) < 0.5
        st(k) = 0;
        continue
    end
    if st(k) == 0 && tmr(k) >= ndead && blk(k) < 0.5
        st(k) = nxt(k); nxt(k) = 3 - nxt(k);
        armed(k) = 0; det(k) = 0; oncnt(k) = 0; tmr(k) = 0;
    end
    if st(k) ~= 0
        if armed(k) < 0.5 && abs(iC(k)) > 5*ithr
            psign(k) = sign(iC(k)); armed(k) = 1;
        end
        if armed(k) > 0.5
            cross = psign(k)*iC(k) < ithr;
        else
            cross = nnom == 0 && abs(iC(k)) < ithr;    % (E28) 무장 전: 부호 없는 영교차
        end
        if cross, det(k) = det(k) + 1; else, det(k) = 0; end
        oncnt(k) = oncnt(k) + 1;
        if (oncnt(k) >= nmin && cross && det(k) > ndet) || oncnt(k) >= nmax ...
                || (nnom > 0 && armed(k) < 0.5 && oncnt(k) >= nnom)
            st(k) = 0; tmr(k) = 0;
        end
    end
    if st(k) == 0
        tmr(k) = tmr(k) + 1;
    end
end

g = zeros(4*N, 1);
for k = 1:N
    b = 4*(k - 1);
    on1 = double(st(k) == 1); on2 = double(st(k) == 2);
    g(b + 1) = on1;    % S1 VIN–A
    g(b + 2) = on2;    % S2 A–V_A
    g(b + 3) = on1;    % S3 V_A–B
    g(b + 4) = on2;    % S4 B–GND
end
st_out = st;
mg_out = [nact; mmode; If; mcancel];
kk = kk + 1;
end

function [hl, nh, rk] = healthy(fl, NM)
% 건전 모듈 목록(번호 순, 앞 nh개가 유효), 개수, 모듈별 순위(고장 모듈은 99)
hl = zeros(NM, 1); rk = 99*ones(NM, 1); nh = 0;
for m = 1:NM
    if fl(m) < 0.5
        nh = nh + 1; hl(nh) = m; rk(m) = nh;
    end
end
end

== matlab function TB32_A25R_ClampMix/Test_Conditions/Profile ==
  data: t input; y output; prm input
function y = prism_tb28_profile(t, prm)
%#codegen
%PRISM_TB28_PROFILE  TB28 시험 조건: TB20의 시험 조건(충전기 전류, 400 V 부하, 48 V 부하, Stage A 위상 동작 여부) + 충전 요청.
%
%   y = prism_tb28_profile(t, prm),   y = [i_ch; Q_400; P_48; en(1:8); chg]  (12×1)
%   prm = [t_I(6) I(6) t_ev mask(8) Q P t_chg_on t_chg_off]  (25개)
%     앞 23개는 prism_tb20_profile과 같다(충전기 전류 구간 선형 6점, 사건 시각, 사건 뒤 위상 동작 여부, 부하 전력).
%     충전 요청 chg = 1(t_chg_on ≤ t < t_chg_off): 차량 충전 제어기가 충전기 전류를 올리기 전에 Stage A 모듈을 모두 켜라고
%     보내는 신호(E28, A25R 요구: 사전 기동 ≥ 600 µs).

y = [prism_tb20_profile(t, prm(1:23)); double(t >= prm(24) && t < prm(25))];
end

== matlab function TB32_A25R_ClampMix/Clamp_Control/VA_Clamp ==
  data: t input; g output; vA input; prm input; st_out output
function [g, st_out] = prism_va_clamp(t, vA, prm)
%#codegen
%PRISM_VA_CLAMP  V_A 노드 클램프(저항 + 스위치) 히스테리시스 비교기. TB20부터.
%
%   [g, st] = prism_va_clamp(t, vA, prm),  prm = [dt v_on v_off n_delay]
%   켬 요청: v_A ≥ v_on, 끔 요청: v_A ≤ v_off(켜진 동안 v_A > v_off이면 유지).
%   요청이 바뀐 뒤 n_delay 간격(스위치·구동 지연, 기본 1 µs) 동안 같은 요청이 이어지면 스위치 상태를 바꾼다.
%   검증 코드 E26(run_event의 클램프)과 같은 논리다.
%   출력: g 게이트(1 켬), st [상태; 지연 카운터]

persistent on cnt want_prev
if isempty(on)
    on = 0; cnt = 0; want_prev = 0;
end
von = prm(2); voff = prm(3); nd = prm(4);
want = double(vA >= von || (on > 0.5 && vA > voff));
if want ~= on
    if want == want_prev
        cnt = cnt + 1;
    else
        cnt = 1;
    end
    if cnt >= nd
        on = want; cnt = 0;
    end
else
    cnt = 0;
end
want_prev = want;
g = on;
st_out = [on; cnt];
end

== matlab function TB32_A25R_ClampMix/Controller_StageC/StageC_Controller ==
  data: t input; u output; meas input; prm input
function u = prism_stageC_reg_ctrl(t, meas, prm)
%#codegen
%PRISM_STAGEC_REG_CTRL  조정형 Stage C(동기 벅 + CLLC DCX) 디지털 제어기. 검증 코드 E22 control(_avg)과 같은 알고리즘.
%
%   표본: T_s = 10 µs(벅 스위칭 주기, 삼각 반송파의 골 = 상측 켜짐 구간 가운데에서 표본 → 인덕터 평균전류).
%   이번 표본에서 계산한 듀티는 다음 표본부터 쓴다(계산 지연 1주기).
%
%   제어 구조(바깥 → 안)
%     출력전류 지령 i_x* = min( 전압 PI(48 V, 교차 1 kHz) + 부하전류 앞먹임,
%                               충전전류 루프: 부하전류 + 충전 제한 + PI(제한 − i_bat)   ← 배터리가 있을 때,
%                               전류 제한: 과도 130 A, 수요가 정격 105 A를 넘은 시간이 2 ms를 넘으면 105 A )
%     인덕터 전류 지령 i_L* = i_x*/n(DCX 전류비)
%     인덕터 전류 PI(교차 5 kHz, 비례항 지령 가중 b) + 중간전압 앞먹임 → 듀티 d = u/v_bus, 0.02 ≤ d ≤ 0.97
%     DCX 보내는 쪽: i_L* > +0.5 A → 1차(V_I → 48 V), < −0.5 A → 2차(48 V → V_I), 그 사이는 유지
%     경부하 두 브리지 구동(prm(25) = P_in > 0일 때, TB15부터): 출력 전력 지령 |i_x*·v_o| < P_in이면 모드 2(두 브리지 같은
%       위상 구동), 모드 2에서 |i_x*·v_o| > P_out(prm(26))이 되면 지령 부호의 보내는 쪽으로 돌아간다. 받는 쪽만 다이오드로 두면
%       역방향 경부하에서 받는 쪽 1차 레그 용량 때문에 DCX 이득이 오른다(검증 코드 E22 gain·both, TB14 사례 F·G).
%   누적 방지: 조건부 적분(포화 방향으로는 적분하지 않음)
%
%   입력  t     시각 [s]
%         meas  [v_bus; i_L; v_I; v_o; i_load; i_bat]  (i_bat: 충전 +, 배터리가 없으면 0)
%         prm   [T_s K_pi K_ii K_pv K_iv I_lim I_rev ff hyst d_max K_pb K_ib I_bat_max I_rated T_OL b  V_ref dt bat_on  I_v0 d0 mode0 iL0 n (P_in P_out (I_i0))]
%               (1–16 = E22 ctl 벡터와 같은 순서, 25·26번이 없으면 두 브리지 구동 안 함(TB14))
%               27번(TB17부터): 전류 PI 적분의 시작값 = (R_L + K_pi(1 − b))·i_L0. 부하가 있는 시작점에서 시작 과도를 없앤다
%               (없으면 0에서 시작: TB14–TB16, 검증 코드 E22와 같음)
%   출력  u     [d; 모드(+1 1차가 보냄, −1 2차가 보냄, 2 두 브리지 구동); i_L 지령 [A]; 선택(0 전압, 1 충전 제한, 2 상한, 3 하한)]

persistent init tn d dn Iv Ii Ib tol mode iref sel
Ts = prm(1); Kpi = prm(2); Kii = prm(3); Kpv = prm(4); Kiv = prm(5);
Ilim = prm(6); Irev = prm(7); ffon = prm(8); hyst = prm(9); dmax = prm(10);
Kpb = prm(11); Kib = prm(12); Ibmax = prm(13); Irated = prm(14); TOL = prm(15); b = prm(16);
Vref = prm(17); dt = prm(18); bat = prm(19); n = prm(24);
Pin = 0; Pout = 0;
if numel(prm) >= 26, Pin = prm(25); Pout = prm(26); end
if isempty(init)
    init = 1; tn = 0; d = prm(21); dn = prm(21); Iv = prm(20); Ii = 0; Ib = 0; tol = 0;
    mode = prm(22); iref = prm(23); sel = 0;
    if numel(prm) >= 27, Ii = prm(27); end
end
if t >= tn - 0.5*dt
    tn = tn + Ts;
    d = dn;                                          % 직전 표본에서 계산한 듀티를 지금부터 적용
    vb = meas(1); iL = meas(2); vI = meas(3); vo = meas(4); iload = meas(5);
    ib = 0;
    if bat > 0.5, ib = meas(6); end
    % ---- 바깥 루프: 출력전류 지령 ---------------------------------------------------------------
    ev = Vref - vo;
    ff = 0;
    if ffon > 0.5, ff = iload; end                   % 앞먹임은 부하전류만(배터리 전류를 넣으면 양의 되먹임)
    ixr = Kpv*ev + Iv + Kiv*ev*Ts + ff;
    sel = 0;
    if bat > 0.5                                     % 충전전류 루프
        eb = Ibmax - ib;
        ixb = iload + Ibmax + Kpb*eb + Ib;
        if ixb < ixr
            ixr = ixb; sel = 1;
            Ib = Ib + Kib*eb*Ts;
        else
            Ib = 0;
        end
    end
    dem = ixr;                                       % 제한 전 수요
    lim = Ilim;
    if tol >= TOL, lim = Irated; end                 % 과부하 시간 제한
    if ixr > lim
        ixr = lim; sel = 2;
    elseif ixr < -Irev
        ixr = -Irev; sel = 3;
    end
    if dem > Irated
        tol = tol + Ts;
    else
        tol = max(0, tol - Ts);
    end
    if sel == 0 || (sel == 2 && ev < 0) || (sel == 3 && ev > 0)
        Iv = Iv + Kiv*ev*Ts;                         % 조건부 적분
    elseif sel == 1
        Iv = min(Iv, ixr - Kpv*ev - ff);             % 충전 제한 중: 전압 적분이 지령을 따라가게
    end
    iref = ixr/n;
    pr = ixr*vo;                                     % 출력 전력 지령
    if Pin > 0 && mode == 2                          % 두 브리지 구동 중: |P*| > P_out이면 보내는 쪽 하나로
        if pr > Pout
            mode = 1;
        elseif pr < -Pout
            mode = -1;
        end
    elseif Pin > 0 && abs(pr) < Pin
        mode = 2;
    elseif iref > hyst
        mode = 1;
    elseif iref < -hyst
        mode = -1;
    end
    % ---- 안쪽 루프: 인덕터 전류 → 듀티 ---------------------------------------------------------------
    ei = iref - iL;
    uu = vI + Kpi*(b*iref - iL) + Ii + Kii*ei*Ts;
    dd = uu/vb;
    if dd > dmax
        dd = dmax;
        if ei < 0, Ii = Ii + Kii*ei*Ts; end
    elseif dd < 0.02
        dd = 0.02;
        if ei > 0, Ii = Ii + Kii*ei*Ts; end
    else
        Ii = Ii + Kii*ei*Ts;
    end
    dn = dd;
end
u = [d; mode; iref; sel];
end

== matlab function TB32_A25R_ClampMix/Gate_StageC/StageC_Gate ==
  data: t input; u input; g output; prm input
function g = prism_gate_stageC_reg(t, u, prm)
%#codegen
%PRISM_GATE_STAGEC_REG  조정형 Stage C 게이트: 동기 벅(중앙 정렬 PWM, 100 kHz) + CLLC DCX(공진점 250 kHz, 보내는 쪽만 스위칭).
%
%   벅: 삼각 반송파 c = 2·min(τ, 1 − τ)(τ = 주기 안 위치, 골 τ = 0에서 제어 표본). 상측은 c < d − t_db/T_b,
%       하측은 c > d + t_db/T_b에서 켠다(전이마다 데드타임 t_db).
%   CLLC: 보내는 쪽 브리지만 [t_dc, T/2) +1(1·4번), [T/2 + t_dc, T) −1(2·3번)으로 스위칭하고, 받는 쪽은 꺼 둔다.
%         데드타임은 보내는 쪽마다 다르다: 1차가 보낼 때 t_dp(자화 전류 수 A로 1차 레그 전이), 2차가 보낼 때 t_ds(전류가 커서
%         전이가 빠르고, 길면 공진전류가 반전해 노드가 되돌아간다. 검증 코드 E22 zvs)
%         (받는 쪽 소자는 역병렬 다이오드로 도통 = 이상 동기정류. 검증 코드 E22 dcx와 같은 방식).
%         보내는 쪽(제어기 출력)은 CLLC 주기 시작에서만 바꿔 반쪽 펄스를 막는다.
%         모드 2(경부하, TB15부터): 두 브리지를 같은 위상으로 구동한다. 1차 데드타임 t_dp, 2차 t_dsb(자화 전류가 두 브리지로
%         나뉘어 2차 전이가 느려지므로 따로 둔다. 검증 코드 E22 both).
%   입력  t    시각 [s]
%         u    [d; 모드(+1 1차가 보냄, −1 2차가 보냄, 2 두 브리지)]
%         prm  [dt T_b t_db T_c t_dp t_ds (t_dsb)]   (7번이 없으면 t_dsb = t_ds)
%   출력  g    [벅 상측 벅 하측 Q1 Q2 Q3 Q4 S1 S2 S3 S4](1 = 켬)

persistent ml
if isempty(ml), ml = 1; end
dt = prm(1); Tb = prm(2); tdb = prm(3); Tc = prm(4); tdp = prm(5); tds = prm(6);
tdsb = tds;
if numel(prm) >= 7, tdsb = prm(7); end
t0 = round(t/dt)*dt;
g = zeros(10, 1);
% ---- 동기 벅 ----------------------------------------------------------------------------------------
tb = mod(t0 + 1e-3*dt, Tb)/Tb;
c = 2*min(tb, 1 - tb);
d = u(1);
g(1) = double(c < d - tdb/Tb);
g(2) = double(c > d + tdb/Tb);
% ---- CLLC DCX ---------------------------------------------------------------------------------------
tau = mod(t0 + 1e-3*dt, Tc);
if tau < dt
    ml = u(2);                                       % 주기 시작에서만 보내는 쪽을 바꾼다
end
sp = double([(tau >= tdp) && (tau < Tc/2); (tau >= Tc/2 + tdp) && (tau < Tc)]);     % 1차 데드타임
ss = double([(tau >= tds) && (tau < Tc/2); (tau >= Tc/2 + tds) && (tau < Tc)]);     % 2차(보낼 때)
sb = double([(tau >= tdsb) && (tau < Tc/2); (tau >= Tc/2 + tdsb) && (tau < Tc)]);   % 2차(두 브리지 구동)
if ml > 1.5                                          % 두 브리지 같은 위상
    g(3:6) = sp([1 2 2 1]);
    g(7:10) = sb([1 2 2 1]);
elseif ml > 0
    g(3:6) = sp([1 2 2 1]);
else
    g(7:10) = ss([1 2 2 1]);
end
end
